simulink model "UAV3_Team_Model"  (R2026b)
settings: Solver=FixedStepDiscrete  StopTime=90  FixedStep=0.1
settings Model: Creator=Ivan  LastModifiedBy=Ivan

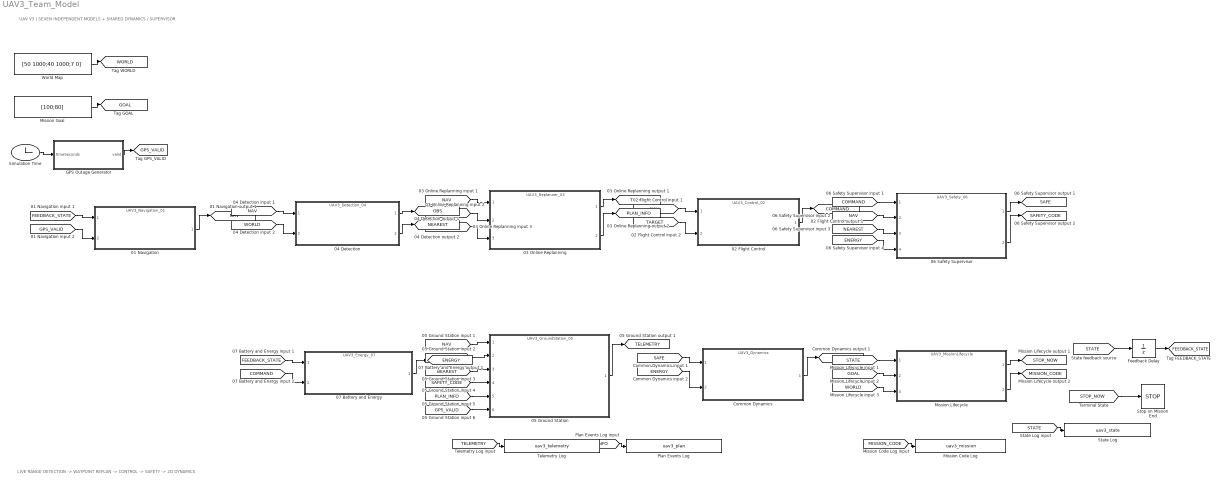
== system UAV3_Team_Model ==
  note: UAV V3 | SEVEN INDEPENDENT MODELS + SHARED DYNAMICS / SUPERVISOR
  note: LIVE RANGE DETECTION -> WAYPOINT REPLAN -> CONTROL -> SAFETY -> 2D DYNAMICS
  01 Navigation : ModelReference  ModelNameDialog=UAV3_Navigation_01  SimulationMode=Normal  ModelReferenceVersion=1.1
  02 Flight Control : ModelReference  ModelNameDialog=UAV3_Control_02  SimulationMode=Normal  ModelReferenceVersion=1.1
  03 Online Replanning : ModelReference  ModelNameDialog=UAV3_Replanner_03  SimulationMode=Normal  ModelReferenceVersion=1.1
  04 Detection : ModelReference  ModelNameDialog=UAV3_Detection_04  SimulationMode=Normal  ModelReferenceVersion=1.1
  05 Ground Station : ModelReference  ModelNameDialog=UAV3_GroundStation_05  SimulationMode=Normal  ModelReferenceVersion=1.1
  06 Safety Supervisor : ModelReference  ModelNameDialog=UAV3_Safety_06  SimulationMode=Normal  ModelReferenceVersion=1.1
  07 Battery and Energy : ModelReference  ModelNameDialog=UAV3_Energy_07  SimulationMode=Normal  ModelReferenceVersion=1.1
  Common Dynamics : ModelReference  ModelNameDialog=UAV3_Dynamics  SimulationMode=Normal  ModelReferenceVersion=1.1
  Feedback Delay : UnitDelay  InitialCondition=[0;0;0;0;100]  SampleTime=0.1
  GPS Outage Generator : MATLAB Function  TreatAsAtomicUnit=on
  Mission Code Log : ToWorkspace  VariableName=uav3_mission  SaveFormat=Timeseries  SampleTime=-1
  Mission Goal : Constant  Value=[100;80]
  Mission Lifecycle : ModelReference  ModelNameDialog=UAV3_MissionLifecycle  SimulationMode=Normal  ModelReferenceVersion=1.1
  Plan Events Log : ToWorkspace  VariableName=uav3_plan  SaveFormat=Timeseries  SampleTime=-1
  Simulation Time : Clock
  State Log : ToWorkspace  VariableName=uav3_state  SaveFormat=Timeseries  SampleTime=-1
  Stop on Mission End : Stop
  Telemetry Log : ToWorkspace  VariableName=uav3_telemetry  SaveFormat=Timeseries  SampleTime=-1
  World Map : Constant  Value=[50 1000;40 1000;7 0]
  tag scope: COMMAND=global, ENERGY=global, FEEDBACK_STATE=global, GOAL=global, GPS_VALID=global, MISSION_CODE=global, NAV=global, NEAREST=global, OBS=global, PLAN_INFO=global, SAFE=global, SAFETY_CODE=global, STATE=global, STOP_NOW=global, TARGET=global, TELEMETRY=global, WORLD=global
  wires:
  World Map/1 -> [WORLD]
  Mission Goal/1 -> [GOAL]
  Simulation Time/1 -> GPS Outage Generator/1(timeSeconds)
  GPS Outage Generator/1(valid) -> [GPS_VALID]
  [FEEDBACK_STATE] -> 01 Navigation/1
  [GPS_VALID] -> 01 Navigation/2
  01 Navigation/1 -> [NAV]
  [NAV] -> 04 Detection/1
  [WORLD] -> 04 Detection/2
  04 Detection/1 -> [OBS]
  04 Detection/2 -> [NEAREST]
  [NAV] -> 03 Online Replanning/1
  [OBS] -> 03 Online Replanning/2
  [GOAL] -> 03 Online Replanning/3
  03 Online Replanning/1 -> [TARGET]
  03 Online Replanning/2 -> [PLAN_INFO]
  [NAV] -> 02 Flight Control/1
  [TARGET] -> 02 Flight Control/2
  02 Flight Control/1 -> [COMMAND]
  [COMMAND] -> 06 Safety Supervisor/1
  [NAV] -> 06 Safety Supervisor/2
  [NEAREST] -> 06 Safety Supervisor/3
  [ENERGY] -> 06 Safety Supervisor/4
  06 Safety Supervisor/1 -> [SAFE]
  06 Safety Supervisor/2 -> [SAFETY_CODE]
  [FEEDBACK_STATE] -> 07 Battery and Energy/1
  [COMMAND] -> 07 Battery and Energy/2
  07 Battery and Energy/1 -> [ENERGY]
  [NAV] -> 05 Ground Station/1
  [ENERGY] -> 05 Ground Station/2
  [NEAREST] -> 05 Ground Station/3
  [SAFETY_CODE] -> 05 Ground Station/4
  [PLAN_INFO] -> 05 Ground Station/5
  [GPS_VALID] -> 05 Ground Station/6
  05 Ground Station/1 -> [TELEMETRY]
  [SAFE] -> Common Dynamics/1
  [ENERGY] -> Common Dynamics/2
  Common Dynamics/1 -> [STATE]
  [STATE] -> Mission Lifecycle/1
  [GOAL] -> Mission Lifecycle/2
  [WORLD] -> Mission Lifecycle/3
  Mission Lifecycle/1 -> [STOP_NOW]
  Mission Lifecycle/2 -> [MISSION_CODE]
  [STATE] -> Feedback Delay/1
  Feedback Delay/1 -> [FEEDBACK_STATE]
  [STATE] -> State Log/1
  [TELEMETRY] -> Telemetry Log/1
  [PLAN_INFO] -> Plan Events Log/1
  [MISSION_CODE] -> Mission Code Log/1
  [STOP_NOW] -> Stop on Mission End/1

== matlab function UAV3_Team_Model/GPS Outage Generator ==
  data: timeSeconds input; valid output
function valid = v3_gps_schedule(timeSeconds)
%V3_GPS_SCHEDULE Synthetic GPS loss between 8 and 10 seconds.
% This is a simulation stimulus, not a physical satellite receiver.
%#codegen
valid=double(timeSeconds<8.0 || timeSeconds>=10.0);
end
